simulink model "IEEE_BUS_68_Baseline"  (R2025a)
settings: Solver=ode23tb  StartTime=0.0  StopTime=150  FixedStep=Ts  MaxStep=0.0001  RelTol=1e-3
PreLoadFcn:
  | PSSMODEL=1;
  | LPSS=0;
  | WAPSS=0;
  | WAPSS2=0;
  | Ts=50e-5;
InitFcn:
  | PSSMODEL=1;
  | LPSS=0;
  | WAPSS=0;
  | WAPSS2=0;
  | Ts=50e-5;
  | 
  | % Required data to 68 Bus benchmark
  | % clear
  | % clc
  | % Definition for the columns
  | % system base =100 MVA
  | 
  | %% Line data Format (line)
  | % All values are given on the same system base MVA
  | % 1: From bus
  | % 2: To bus
  | % 3: Resistance (pu)
  | % 4: Reactance  (pu)
  | % 5: Charge     (pu)
  | % 6: Transformer Tap Amplitute
  | % 7: base MVA
  | % 8: Nomonal Voltage (KV)
  | 
  | %1   2    3        4       5       6        7      8
  | line=[...
  | 1	54	0	     0.0181	  0	      1.025     100    13.8
  | 2	58	0	     0.025	  0	      1.070     100    13.8
  | 3	62	0	     0.02	  0	      1.070     100    13.8
  | 4	19	0.0007	 0.0142	  0	      1.070     100    13.8
  | 5	20	0.0009	 0.018	  0	      1.009     100    13.8
  | 6	22	0	     0.0143	  0	      1.025     100    13.8
  | 7	23	0.0005	 0.0272	  0	      0         100    13.8
  | 8	25	0.0006	 0.0232	  0	      1.025     100    13.8
  | 9	29	0.0008	 0.0156   0	      1.025     100    13.8
  | 10	31	0	     0.026	  0	      1.04      100    13.8
  | 11	32	0	     0.013	  0	      1.04      100    13.8
  | 12	36	0	     0.0075	  0	      1.04      100    13.8
  | 13	17	0	     0.0033	  0	      1.04      100    13.8
  | 14	41	0	     0.0015	  0	      1         100    13.8
  | 15	42	0	     0.0015	  0	      1         100    13.8
  | 16	18	0	     0.003	  0	      1         100    13.8
  | 17	36	0.0005	 0.0045	  0.32	  0         100    138
  | 17	43	0.0005	 0.0276	  0	      0         100    138
  | 18	42	0.004	 0.06	  2.25    0         100    138
  | 18	49	0.0076	 0.1141	  1.16    0	        100    138
  | 18	50	0.0012	 0.0288	  2.06	  0         100    138
  | 20	19	0.0007	 0.0138	  0       1.06	    100    138
  | 19	68	0.0016	 0.0195	  0.304	  0         100    138
  | 21	22	0.0008	 0.014	  0.2565  0	        100    138
  | 21	68	0.0008	 0.0135	  0.2548  0	        100    138
  | 22	23	0.0006	 0.0096	  0.1846  0	        100    138
  | 23	24	0.0022	 0.035	  0.361	  0         100    138
  | 24	68	0.0003	 0.0059	  0.068	  0         100    138
  | 25	26	0.0032	 0.0323	  0.531	  0         100    138
  | 25	54	0.007	 0.0086	  0.146	  0         100    138
  | 26	27	0.0014	 0.0147	  0.2396  0	        100    138
  | 26	28	0.0043	 0.0474	  0.7802  0	        100    138
  | 26	29	0.0057	 0.0625	  1.029	  0         100    138
  | 27	37	0.0013	 0.0173	  0.3216  0	        100    138
  | 27	53	0.032	 0.32	  0.41	  0         100    138
  | ... (+206 lines)
undefined symbols (not defined in the file or in its folder): D1, Delta
libraries: spsRMSLib x73, spsThreePhaseVIMeasurementLib x69, spsLoadFlowBusLib x69, spsThreePhasePISectionLineLib x64, spsThreePhaseParallelRLCLoadLib x35, spsGenericPowerSystemStabilizerLib x32, spsThreePhaseSeriesRLCLoadLib x21, spsThreePhaseTransformerTwoWindingsLib x21, spsSynchronousMachinepuStandardLib x19, spsExcitationSystemLib x16, spsMultiBandPowerSystemStabilizerLib x16, spsSteamTurbineandGovernorLib x16
(part 6 of 7)

== system IEEE_BUS_68_Baseline/area-2/gen3/M3: Turbine & Regulators  ==
  note: M3
  m3 : Inport
  Pref3 : Inport  Port=2
  Vref3 : Inport  Port=3
  PSS3 : Inport  Port=4
  Bus Selector : BusSelector  OutputSignals="Mechanical.Rotor speed  wm  (pu),Mechanical.Rotor angle deviation  d_theta (rad),Mechanical.Electrical power  Pe (pu),Mechanical.Rotor speed deviation  dw (pu),Mechanical.Rotor mechanical angle  theta (deg),dq0 components.Stator voltage  vd (pu),dq0 components.Stator voltage  vq (pu),Output reactive power  Qeo (pu)"
  "Delta Pa PSS 3 " : spsGenericPowerSystemStabilizerLib/Generic Power System Stabilizer  Tsensor=15e-3  K=2.5*1.25  Twashout=1  Tleadlag1=[60e-3 1]  Tleadlag2=[0 0]  VSlimits=[-0.15 0.15]  Vinit=0  Plot_On=off  MagdB_On=on  FreqRange=logspace(-2,2,500)
      settings: LibrarySourceBlock=|
      | sps_lib/Electrical Machines/Synchronous Machine Control/Generic
      | Power System Stabilizer
  Delta w PSS (Kundur) 3 : spsGenericPowerSystemStabilizerLib/Generic Power System Stabilizer  Tsensor=15e-3  K=30  Twashout=10  Tleadlag1=[50e-3 20e-3]  Tleadlag2=[3 5.4]  VSlimits=[-0.15 0.15]  Vinit=0  Plot_On=off  MagdB_On=on  FreqRange=logspace(-2,2,500)
      settings: LibrarySourceBlock=|
      | sps_lib/Electrical Machines/Synchronous Machine Control/Generic
      | Power System Stabilizer
  EXCITATION3 : spsExcitationSystemLib/Excitation System  tr=AVR_Data(3,1)  reg=[ AVR_Data(3,2:3) ]  exc=[ 1, 0 ]  tgr=[ AVR_Data(3,4:5)]  damp=[ 0, 0 ]  sat=[ 0, 0 ]  lim="[ AVR_Data(3,7:8)  0 ]"  v0=[0.983 0.98901]
      settings: LibrarySourceBlock=sps_lib/Electrical Machines/Synchronous Machine Control/Excitation System
  MB-PSS3 : spsMultiBandPowerSystemStabilizerLib/Multi-Band Power System Stabilizer  OperationMode=Simplified settings  Kg=MB(1)  GL=[MB(2) MB(3)]  GI=[MB(4) MB(5)]  GH=[MB(6) MB(7)]  GLd=[66 66 9.4]  TcLF=[1.667 2 0 0 0 0 2 2.4 0 0 0 0 1 1]  GId=[66 66 47.6]  TcIF=[1 1 0.25 0.3 0 0 1 1 0.3 0.36 0 0 0 0]  GHd=[66 66 233]  TcHF="[0.01 0.012 0 0 0 0  0.012 0.0144 0 0 0 0 1 1]"  LIM=[.075 .15 .15 .15]  Plot_On=off  MagdB_On=off  FreqRange=logspace(-2,2,500)
      settings: LibrarySourceBlock=|
      | sps_lib/Electrical Machines/Synchronous Machine Control/Multi-Band
      | Power System Stabilizer
  Multiport Switch1 : MultiPortSwitch  Inputs=4  SaturateOnIntegerOverflow=off
  PSS model3 : Constant  Value=0
  PSS model4 : Constant
  Real-Imag to Complex1 : RealImagToComplex
  STG3 : spsSteamTurbineandGovernorLib/Steam Turbine and Governor  gentype=Tandem-compound (single mass)  reg1="[ 1  0.05    0 ]"  reg2="[ 0.001  0.15 ]"  reg3="[ -0.1  0.1  0  4.496 ]"  N=Ns  turb1="[ 0  10   3.3   0.5   ]"  turb2="[   0   0.36    0.36   0.28   ]"  HA="[ 0.046  1.430  1.465   0.192 ]"  KA="[ 90.44  53.88  64.59   62.94  ]"  DA="[ 0.0115  0.3575  0.3663   0.0137  ]"  ini1=0.325  ini2=[0.779316,-31.4247]
      settings: LibrarySourceBlock=|
      | sps_lib/Electrical Machines/Synchronous Machine Control/Steam Turbine
      | and Governor
  Sum2 : Sum  InputSameDT=on  SaturateOnIntegerOverflow=on  OutDataTypeStr=Inherit: Same as first input
  Sum3 : Sum  Inputs=-+  InputSameDT=on  SaturateOnIntegerOverflow=on  OutDataTypeStr=Inherit: Same as first input
  Terminator3 : Terminator
  Terminator4 : Terminator
  Terminator5 : Terminator
  wref3 : Constant
  Pm3 : Outport  InitialOutput=0
  Vf3 : Outport  Port=2  InitialOutput=0
  tag scope: EFD3=global, Pa3=global, Pe3=global, Q3=global, Vt3=global, d_theta3=global, pss3=global, theta3=global, w3=global
  wires:
  PSS3/1 -> Sum2/1
  Multiport Switch1/1 -> EXCITATION3/4, [pss3]
  PSS model3/1 -> Multiport Switch1/2
  MB-PSS3/1 -> Multiport Switch1/3
  Delta w PSS (Kundur) 3/1 -> Multiport Switch1/4
  "Delta Pa PSS 3 "/1 -> Multiport Switch1/5
  PSS model4/1 -> Sum2/2
  Sum2/1 -> Multiport Switch1/1
  Sum3/1 -> "Delta Pa PSS 3 "/1, [Pa3]  "Pm-Pe"
  Bus Selector/8 -> [Q3]  "<Output reactive power  Qeo (pu)>"
  Bus Selector/4 -> MB-PSS3/1, Delta w PSS (Kundur) 3/1  "<Rotor speed deviation  dw (pu)>"
  Bus Selector/3 -> [Pe3], Sum3/1  "<Electrical power  Pe (pu)>"
  Bus Selector/2 -> [d_theta3], STG3/4  "<Rotor angle deviation  d_theta (rad)>"
  Bus Selector/1 -> STG3/3, [w3]  "<Rotor speed  wm  (pu)>"
  STG3/1 -> Terminator5/1
  STG3/2 -> Terminator4/1
  STG3/4 -> Pm3/1, Sum3/2
  STG3/3 -> Terminator3/1
  Bus Selector/6 -> Real-Imag to Complex1/1, EXCITATION3/2  "<Stator voltage  vd (pu)>"
  Bus Selector/5 -> [theta3]  "<Rotor mechanical angle  theta (deg)>"
  Real-Imag to Complex1/1 -> [Vt3]
  EXCITATION3/1 -> [EFD3], Vf3/1
  Vref3/1 -> EXCITATION3/1
  m3/1 -> Bus Selector/1
  Pref3/1 -> STG3/2
  wref3/1 -> STG3/1
  Bus Selector/7 -> Real-Imag to Complex1/2, EXCITATION3/3  "<Stator voltage  vq (pu)>"

== system IEEE_BUS_68_Baseline/area-3/G1/M1: Turbine & Regulators  ==
  note: M1
  m1 : Inport
  Pref1 : Inport  Port=2
  Vref1 : Inport  Port=3
  PSS1 : Inport  Port=4
  Bus Selector : BusSelector  OutputSignals="Mechanical.Rotor speed  wm  (pu),Mechanical.Rotor angle deviation  d_theta (rad),Mechanical.Electrical power  Pe (pu),Mechanical.Rotor speed deviation  dw (pu),Mechanical.Rotor mechanical angle  theta (deg),dq0 components.Stator voltage  vd (pu),dq0 components.Stator voltage  vq (pu),Output reactive power  Qeo (pu)"
  "Delta Pa PSS 1 " : spsGenericPowerSystemStabilizerLib/Generic Power System Stabilizer  Tsensor=15e-3  K=2.5*1.25  Twashout=1  Tleadlag1=[60e-3 1]  Tleadlag2=[0 0]  VSlimits=[-0.15 0.15]  Vinit=0  Plot_On=off  MagdB_On=on  FreqRange=logspace(-2,2,500)
      settings: LibrarySourceBlock=|
      | sps_lib/Electrical Machines/Synchronous Machine Control/Generic
      | Power System Stabilizer
  Delta w PSS (Kundur) 1 : spsGenericPowerSystemStabilizerLib/Generic Power System Stabilizer  Tsensor=15e-3  K=30  Twashout=10  Tleadlag1=[50e-3 20e-3]  Tleadlag2=[3 5.4]  VSlimits=[-0.15 0.15]  Vinit=0  Plot_On=off  MagdB_On=on  FreqRange=logspace(-2,2,500)
      settings: LibrarySourceBlock=|
      | sps_lib/Electrical Machines/Synchronous Machine Control/Generic
      | Power System Stabilizer
  EXCITATION1 : spsExcitationSystemLib/Excitation System  tr=AVR_Data(1,1)  reg=[ AVR_Data(1,2:3) ]  exc=[ 1, 0 ]  tgr=[ AVR_Data(1,4:5)]  damp=[ 0, 0 ]  sat=[ 0, 0 ]  lim="[ AVR_Data(1,7:8)  0 ]"  v0=[1.045 1.06]
      settings: LibrarySourceBlock=sps_lib/Electrical Machines/Synchronous Machine Control/Excitation System
  MB-PSS1 : spsMultiBandPowerSystemStabilizerLib/Multi-Band Power System Stabilizer  OperationMode=Simplified settings  Kg=MB(1)  GL=[MB(2) MB(3)]  GI=[MB(4) MB(5)]  GH=[MB(6) MB(7)]  GLd=[66 66 9.4]  TcLF=[1.667 2 0 0 0 0 2 2.4 0 0 0 0 1 1]  GId=[66 66 47.6]  TcIF=[1 1 0.25 0.3 0 0 1 1 0.3 0.36 0 0 0 0]  GHd=[66 66 233]  TcHF="[0.01 0.012 0 0 0 0  0.012 0.0144 0 0 0 0 1 1]"  LIM=[.075 .15 .15 .15]  Plot_On=off  MagdB_On=off  FreqRange=logspace(-2,2,500)
      settings: LibrarySourceBlock=|
      | sps_lib/Electrical Machines/Synchronous Machine Control/Multi-Band
      | Power System Stabilizer
  Multiport Switch1 : MultiPortSwitch  Inputs=4  SaturateOnIntegerOverflow=off
  PSS model3 : Constant  Value=0
  PSS model4 : Constant
  Real-Imag to Complex1 : RealImagToComplex
  STG1 : spsSteamTurbineandGovernorLib/Steam Turbine and Governor  gentype=Tandem-compound (single mass)  reg1="[ 1  0.05    0 ]"  reg2="[ 0.001  0.15 ]"  reg3="[ -0.1  0.1  0  4.496 ]"  N=Ns  turb1="[ 0  10   3.3   0.5   ]"  turb2="[   0   0.36    0.36   0.28   ]"  HA="[ 0.046  1.430  1.465   0.192 ]"  KA="[ 90.44  53.88  64.59   62.94  ]"  DA="[ 0.0115  0.3575  0.3663   0.0137  ]"  ini1=0.25  ini2=[0.779316,-31.4247]
      settings: LibrarySourceBlock=|
      | sps_lib/Electrical Machines/Synchronous Machine Control/Steam Turbine
      | and Governor
  Sum2 : Sum  InputSameDT=on  SaturateOnIntegerOverflow=on  OutDataTypeStr=Inherit: Same as first input
  Sum3 : Sum  Inputs=-+  InputSameDT=on  SaturateOnIntegerOverflow=on  OutDataTypeStr=Inherit: Same as first input
  Terminator3 : Terminator
  Terminator4 : Terminator
  Terminator5 : Terminator
  wref1 : Constant
  Pm1 : Outport  InitialOutput=0
  Vf1 : Outport  Port=2  InitialOutput=0
  tag scope: EFD1=global, Pa1=global, Pe1=global, Q1=global, Vt1=global, d_theta1=global, pss1=global, theta1=global, w1=global
  wires:
  PSS1/1 -> Sum2/1
  Multiport Switch1/1 -> EXCITATION1/4, [pss1]
  PSS model3/1 -> Multiport Switch1/2
  MB-PSS1/1 -> Multiport Switch1/3
  Delta w PSS (Kundur) 1/1 -> Multiport Switch1/4
  "Delta Pa PSS 1 "/1 -> Multiport Switch1/5
  PSS model4/1 -> Sum2/2
  Sum2/1 -> Multiport Switch1/1
  Sum3/1 -> "Delta Pa PSS 1 "/1, [Pa1]  "Pm-Pe"
  Bus Selector/8 -> [Q1]  "<Output reactive power  Qeo (pu)>"
  Bus Selector/4 -> MB-PSS1/1, Delta w PSS (Kundur) 1/1  "<Rotor speed deviation  dw (pu)>"
  Bus Selector/3 -> [Pe1], Sum3/1  "<Electrical power  Pe (pu)>"
  Bus Selector/2 -> [d_theta1], STG1/4  "<Rotor angle deviation  d_theta (rad)>"
  Bus Selector/1 -> STG1/3, [w1]  "<Rotor speed  wm  (pu)>"
  STG1/1 -> Terminator5/1
  STG1/2 -> Terminator4/1
  STG1/4 -> Pm1/1, Sum3/2
  STG1/3 -> Terminator3/1
  Bus Selector/6 -> Real-Imag to Complex1/1, EXCITATION1/2  "<Stator voltage  vd (pu)>"
  Bus Selector/5 -> [theta1]  "<Rotor mechanical angle  theta (deg)>"
  Real-Imag to Complex1/1 -> [Vt1]
  EXCITATION1/1 -> [EFD1], Vf1/1
  Vref1/1 -> EXCITATION1/1
  m1/1 -> Bus Selector/1
  Pref1/1 -> STG1/2
  wref1/1 -> STG1/1
  Bus Selector/7 -> Real-Imag to Complex1/2, EXCITATION1/3  "<Stator voltage  vq (pu)>"

== system IEEE_BUS_68_Baseline/area-3/G8/M8: Turbine & Regulators  ==
  note: M8
  m8 : Inport
  Pref8 : Inport  Port=2
  Vref8 : Inport  Port=3
  PSS8 : Inport  Port=4
  Bus Selector : BusSelector  OutputSignals="Mechanical.Rotor speed  wm  (pu),Mechanical.Rotor angle deviation  d_theta (rad),Mechanical.Electrical power  Pe (pu),Mechanical.Rotor speed deviation  dw (pu),Mechanical.Rotor mechanical angle  theta (deg),dq0 components.Stator voltage  vd (pu),dq0 components.Stator voltage  vq (pu),Output reactive power  Qeo (pu)"
  "Delta Pa PSS 8 " : spsGenericPowerSystemStabilizerLib/Generic Power System Stabilizer  Tsensor=15e-3  K=2.5*1.25  Twashout=1  Tleadlag1=[60e-3 1]  Tleadlag2=[0 0]  VSlimits=[-0.15 0.15]  Vinit=0  Plot_On=off  MagdB_On=on  FreqRange=logspace(-2,2,500)
      settings: LibrarySourceBlock=|
      | sps_lib/Electrical Machines/Synchronous Machine Control/Generic
      | Power System Stabilizer
  Delta w PSS (Kundur) 8 : spsGenericPowerSystemStabilizerLib/Generic Power System Stabilizer  Tsensor=15e-3  K=30  Twashout=10  Tleadlag1=[50e-3 20e-3]  Tleadlag2=[3 5.4]  VSlimits=[-0.15 0.15]  Vinit=0  Plot_On=off  MagdB_On=on  FreqRange=logspace(-2,2,500)
      settings: LibrarySourceBlock=|
      | sps_lib/Electrical Machines/Synchronous Machine Control/Generic
      | Power System Stabilizer
  EXCITATION8 : spsExcitationSystemLib/Excitation System  tr=AVR_Data(8,1)  reg=[ AVR_Data(8,2:3) ]  exc=[ 1, 0 ]  tgr=[ AVR_Data(8,4:5)]  damp=[ 0, 0 ]  sat=[ 0, 0 ]  lim="[ AVR_Data(8,7:8)  0 ]"  v0=[1.03 1.0424]
      settings: LibrarySourceBlock=sps_lib/Electrical Machines/Synchronous Machine Control/Excitation System
  MB-PSS8 : spsMultiBandPowerSystemStabilizerLib/Multi-Band Power System Stabilizer  OperationMode=Simplified settings  Kg=MB(1)  GL=[MB(2) MB(3)]  GI=[MB(4) MB(5)]  GH=[MB(6) MB(7)]  GLd=[66 66 9.4]  TcLF=[1.667 2 0 0 0 0 2 2.4 0 0 0 0 1 1]  GId=[66 66 47.6]  TcIF=[1 1 0.25 0.3 0 0 1 1 0.3 0.36 0 0 0 0]  GHd=[66 66 233]  TcHF="[0.01 0.012 0 0 0 0  0.012 0.0144 0 0 0 0 1 1]"  LIM=[.075 .15 .15 .15]  Plot_On=off  MagdB_On=off  FreqRange=logspace(-2,2,500)
      settings: LibrarySourceBlock=|
      | sps_lib/Electrical Machines/Synchronous Machine Control/Multi-Band
      | Power System Stabilizer
  Multiport Switch1 : MultiPortSwitch  Inputs=4  SaturateOnIntegerOverflow=off
  PSS model3 : Constant  Value=0
  PSS model4 : Constant
  Real-Imag to Complex1 : RealImagToComplex
  STG8 : spsSteamTurbineandGovernorLib/Steam Turbine and Governor  gentype=Tandem-compound (single mass)  reg1="[ 1  0.05    0 ]"  reg2="[ 0.001  0.15 ]"  reg3="[ -0.1  0.1  0  4.496 ]"  N=Ns  turb1="[ 0  10   3.3   0.5   ]"  turb2="[   0   0.36    0.36   0.28   ]"  HA="[ 0.046  1.430  1.465   0.192 ]"  KA="[ 90.44  53.88  64.59   62.94  ]"  DA="[ 0.0115  0.3575  0.3663   0.0137  ]"  ini1=0.54  ini2=[0.779316,-31.4247]
      settings: LibrarySourceBlock=|
      | sps_lib/Electrical Machines/Synchronous Machine Control/Steam Turbine
      | and Governor
  Sum2 : Sum  InputSameDT=on  SaturateOnIntegerOverflow=on  OutDataTypeStr=Inherit: Same as first input
  Sum3 : Sum  Inputs=-+  InputSameDT=on  SaturateOnIntegerOverflow=on  OutDataTypeStr=Inherit: Same as first input
  Terminator3 : Terminator
  Terminator4 : Terminator
  Terminator5 : Terminator
  wref8 : Constant
  Pm8 : Outport  InitialOutput=0
  Vf8 : Outport  Port=2  InitialOutput=0
  tag scope: EFD8=global, Pa8=global, Pe8=global, Q8=global, Vt8=global, d_theta8=global, pss8=global, theta8=global, w8=global
  wires:
  Bus Selector/7 -> EXCITATION8/3, Real-Imag to Complex1/2  "<Stator voltage  vq (pu)>"
  wref8/1 -> STG8/1
  Pref8/1 -> STG8/2
  m8/1 -> Bus Selector/1
  Vref8/1 -> EXCITATION8/1
  EXCITATION8/1 -> Vf8/1, [EFD8]
  Real-Imag to Complex1/1 -> [Vt8]
  Bus Selector/5 -> [theta8]  "<Rotor mechanical angle  theta (deg)>"
  Bus Selector/6 -> EXCITATION8/2, Real-Imag to Complex1/1  "<Stator voltage  vd (pu)>"
  STG8/3 -> Terminator3/1
  STG8/4 -> Sum3/2, Pm8/1
  STG8/2 -> Terminator4/1
  STG8/1 -> Terminator5/1
  Bus Selector/1 -> [w8], STG8/3  "<Rotor speed  wm  (pu)>"
  Bus Selector/2 -> STG8/4, [d_theta8]  "<Rotor angle deviation  d_theta (rad)>"
  Bus Selector/3 -> Sum3/1, [Pe8]  "<Electrical power  Pe (pu)>"
  Bus Selector/4 -> Delta w PSS (Kundur) 8/1, MB-PSS8/1  "<Rotor speed deviation  dw (pu)>"
  Bus Selector/8 -> [Q8]  "<Output reactive power  Qeo (pu)>"
  Sum3/1 -> [Pa8], "Delta Pa PSS 8 "/1  "Pm-Pe"
  Sum2/1 -> Multiport Switch1/1
  PSS model4/1 -> Sum2/2
  "Delta Pa PSS 8 "/1 -> Multiport Switch1/5
  Delta w PSS (Kundur) 8/1 -> Multiport Switch1/4
  MB-PSS8/1 -> Multiport Switch1/3
  PSS model3/1 -> Multiport Switch1/2
  Multiport Switch1/1 -> [pss8], EXCITATION8/4
  PSS8/1 -> Sum2/1

== system IEEE_BUS_68_Baseline/area-3/G9/M9: Turbine & Regulators  ==
  note: M9
  m9 : Inport
  Pref9 : Inport  Port=2
  Vref9 : Inport  Port=3
  PSS9 : Inport  Port=4
  Bus Selector : BusSelector  OutputSignals="Mechanical.Rotor speed  wm  (pu),Mechanical.Rotor angle deviation  d_theta (rad),Mechanical.Electrical power  Pe (pu),Mechanical.Rotor speed deviation  dw (pu),Mechanical.Rotor mechanical angle  theta (deg),dq0 components.Stator voltage  vd (pu),dq0 components.Stator voltage  vq (pu),Output reactive power  Qeo (pu)"
  "Delta Pa PSS 9 " : spsGenericPowerSystemStabilizerLib/Generic Power System Stabilizer  Tsensor=15e-3  K=2.5*1.25  Twashout=1  Tleadlag1=[60e-3 1]  Tleadlag2=[0 0]  VSlimits=[-0.15 0.15]  Vinit=0  Plot_On=off  MagdB_On=on  FreqRange=logspace(-2,2,500)
      settings: LibrarySourceBlock=|
      | sps_lib/Electrical Machines/Synchronous Machine Control/Generic
      | Power System Stabilizer
  Delta w PSS (Kundur) 9 : spsGenericPowerSystemStabilizerLib/Generic Power System Stabilizer  Tsensor=15e-3  K=30  Twashout=10  Tleadlag1=[50e-3 20e-3]  Tleadlag2=[3 5.4]  VSlimits=[-0.15 0.15]  Vinit=0  Plot_On=off  MagdB_On=on  FreqRange=logspace(-2,2,500)
      settings: LibrarySourceBlock=|
      | sps_lib/Electrical Machines/Synchronous Machine Control/Generic
      | Power System Stabilizer
  EXCITATION9 : spsExcitationSystemLib/Excitation System  tr=AVR_Data(9,1)  reg=[ AVR_Data(9,2:3) ]  exc=[ 1, 0 ]  tgr=[ AVR_Data(9,4:5)]  damp=[ 0, 0 ]  sat=[ 0, 0 ]  lim="[ AVR_Data(9,7:8)  0 ]"  v0=[1.025 1.0447]
      settings: LibrarySourceBlock=sps_lib/Electrical Machines/Synchronous Machine Control/Excitation System
  MB-PSS9 : spsMultiBandPowerSystemStabilizerLib/Multi-Band Power System Stabilizer  OperationMode=Simplified settings  Kg=MB(1)  GL=[MB(2) MB(3)]  GI=[MB(4) MB(5)]  GH=[MB(6) MB(7)]  GLd=[66 66 9.4]  TcLF=[1.667 2 0 0 0 0 2 2.4 0 0 0 0 1 1]  GId=[66 66 47.6]  TcIF=[1 1 0.25 0.3 0 0 1 1 0.3 0.36 0 0 0 0]  GHd=[66 66 233]  TcHF="[0.01 0.012 0 0 0 0  0.012 0.0144 0 0 0 0 1 1]"  LIM=[.075 .15 .15 .15]  Plot_On=off  MagdB_On=off  FreqRange=logspace(-2,2,500)
      settings: LibrarySourceBlock=|
      | sps_lib/Electrical Machines/Synchronous Machine Control/Multi-Band
      | Power System Stabilizer
  Multiport Switch1 : MultiPortSwitch  Inputs=4  SaturateOnIntegerOverflow=off
  PSS model3 : Constant  Value=0
  PSS model4 : Constant
  Real-Imag to Complex1 : RealImagToComplex
  STG9 : spsSteamTurbineandGovernorLib/Steam Turbine and Governor  gentype=Tandem-compound (single mass)  reg1="[ 1  0.05    0 ]"  reg2="[ 0.001  0.15 ]"  reg3="[ -0.1  0.1  0  4.496 ]"  N=Ns  turb1="[ 0  10   3.3   0.5   ]"  turb2="[   0   0.36    0.36   0.28   ]"  HA="[ 0.046  1.430  1.465   0.192 ]"  KA="[ 90.44  53.88  64.59   62.94  ]"  DA="[ 0.0115  0.3575  0.3663   0.0137  ]"  ini1=0.8  ini2=[0.779316,-31.4247]
      settings: LibrarySourceBlock=|
      | sps_lib/Electrical Machines/Synchronous Machine Control/Steam Turbine
      | and Governor
  Sum2 : Sum  InputSameDT=on  SaturateOnIntegerOverflow=on  OutDataTypeStr=Inherit: Same as first input
  Sum3 : Sum  Inputs=-+  InputSameDT=on  SaturateOnIntegerOverflow=on  OutDataTypeStr=Inherit: Same as first input
  Terminator3 : Terminator
  Terminator4 : Terminator
  Terminator5 : Terminator
  wref9 : Constant
  Pm9 : Outport  InitialOutput=0
  Vf9 : Outport  Port=2  InitialOutput=0
  tag scope: EFD9=global, Pa9=global, Pe9=global, Q9=global, Vt9=global, d_theta9=global, pss9=global, theta9=global, w9=global
  wires:
  PSS9/1 -> Sum2/1
  Multiport Switch1/1 -> EXCITATION9/4, [pss9]
  PSS model3/1 -> Multiport Switch1/2
  MB-PSS9/1 -> Multiport Switch1/3
  Delta w PSS (Kundur) 9/1 -> Multiport Switch1/4
  "Delta Pa PSS 9 "/1 -> Multiport Switch1/5
  PSS model4/1 -> Sum2/2
  Sum2/1 -> Multiport Switch1/1
  Sum3/1 -> "Delta Pa PSS 9 "/1, [Pa9]  "Pm-Pe"
  Bus Selector/8 -> [Q9]  "<Output reactive power  Qeo (pu)>"
  Bus Selector/4 -> MB-PSS9/1, Delta w PSS (Kundur) 9/1  "<Rotor speed deviation  dw (pu)>"
  Bus Selector/3 -> [Pe9], Sum3/1  "<Electrical power  Pe (pu)>"
  Bus Selector/2 -> [d_theta9], STG9/4  "<Rotor angle deviation  d_theta (rad)>"
  Bus Selector/1 -> STG9/3, [w9]  "<Rotor speed  wm  (pu)>"
  STG9/1 -> Terminator5/1
  STG9/2 -> Terminator4/1
  STG9/4 -> Pm9/1, Sum3/2
  STG9/3 -> Terminator3/1
  Bus Selector/6 -> Real-Imag to Complex1/1, EXCITATION9/2  "<Stator voltage  vd (pu)>"
  Bus Selector/5 -> [theta9]  "<Rotor mechanical angle  theta (deg)>"
  Real-Imag to Complex1/1 -> [Vt9]
  EXCITATION9/1 -> [EFD9], Vf9/1
  Vref9/1 -> EXCITATION9/1
  m9/1 -> Bus Selector/1
  Pref9/1 -> STG9/2
  wref9/1 -> STG9/1
  Bus Selector/7 -> Real-Imag to Complex1/2, EXCITATION9/3  "<Stator voltage  vq (pu)>"

== system IEEE_BUS_68_Baseline/area-4/G10/M10: Turbine & Regulators  ==
  note: M10
  m10 : Inport
  Pref10 : Inport  Port=2
  Vref10 : Inport  Port=3
  PSS10 : Inport  Port=4
  Bus Selector : BusSelector  OutputSignals="Mechanical.Rotor speed  wm  (pu),Mechanical.Rotor angle deviation  d_theta (rad),Mechanical.Electrical power  Pe (pu),Mechanical.Rotor speed deviation  dw (pu),Mechanical.Rotor mechanical angle  theta (deg),dq0 components.Stator voltage  vd (pu),dq0 components.Stator voltage  vq (pu),Output reactive power  Qeo (pu)"
  "Delta Pa PSS 10 " : spsGenericPowerSystemStabilizerLib/Generic Power System Stabilizer  Tsensor=15e-3  K=2.5*1.25  Twashout=1  Tleadlag1=[60e-3 1]  Tleadlag2=[0 0]  VSlimits=[-0.15 0.15]  Vinit=0  Plot_On=off  MagdB_On=on  FreqRange=logspace(-2,2,500)
      settings: LibrarySourceBlock=|
      | sps_lib/Electrical Machines/Synchronous Machine Control/Generic
      | Power System Stabilizer
  Delta w PSS (Kundur) 10 : spsGenericPowerSystemStabilizerLib/Generic Power System Stabilizer  Tsensor=15e-3  K=30  Twashout=10  Tleadlag1=[50e-3 20e-3]  Tleadlag2=[3 5.4]  VSlimits=[-0.15 0.15]  Vinit=0  Plot_On=off  MagdB_On=on  FreqRange=logspace(-2,2,500)
      settings: LibrarySourceBlock=|
      | sps_lib/Electrical Machines/Synchronous Machine Control/Generic
      | Power System Stabilizer
  EXCITATION10 : spsExcitationSystemLib/Excitation System  tr=AVR_Data(7,1)  reg=[ AVR_Data(7,2:3) ]  exc=[ 1, 0 ]  tgr=[ AVR_Data(7,4:5)]  damp=[ 0, 0 ]  sat=[ 0, 0 ]  lim="[ AVR_Data(7,7:8)  0 ]"  v0=[1.01 1.0155]
      settings: LibrarySourceBlock=sps_lib/Electrical Machines/Synchronous Machine Control/Excitation System
  MB-PSS10 : spsMultiBandPowerSystemStabilizerLib/Multi-Band Power System Stabilizer  OperationMode=Simplified settings  Kg=MB(1)  GL=[MB(2) MB(3)]  GI=[MB(4) MB(5)]  GH=[MB(6) MB(7)]  GLd=[66 66 9.4]  TcLF=[1.667 2 0 0 0 0 2 2.4 0 0 0 0 1 1]  GId=[66 66 47.6]  TcIF=[1 1 0.25 0.3 0 0 1 1 0.3 0.36 0 0 0 0]  GHd=[66 66 233]  TcHF="[0.01 0.012 0 0 0 0  0.012 0.0144 0 0 0 0 1 1]"  LIM=[.075 .15 .15 .15]  Plot_On=off  MagdB_On=off  FreqRange=logspace(-2,2,500)
      settings: LibrarySourceBlock=|
      | sps_lib/Electrical Machines/Synchronous Machine Control/Multi-Band
      | Power System Stabilizer
  Multiport Switch1 : MultiPortSwitch  Inputs=4  SaturateOnIntegerOverflow=off
  PSS model3 : Constant  Value=0
  PSS model4 : Constant
  Real-Imag to Complex1 : RealImagToComplex
  STG10 : spsSteamTurbineandGovernorLib/Steam Turbine and Governor  gentype=Tandem-compound (single mass)  reg1="[ 1  0.05    0 ]"  reg2="[ 0.001  0.15 ]"  reg3="[ -0.1  0.1  0  4.496 ]"  N=Ns  turb1="[ 0  10   3.3   0.5   ]"  turb2="[   0   0.36    0.36   0.28   ]"  HA="[ 0.046  1.430  1.465   0.192 ]"  KA="[ 90.44  53.88  64.59   62.94  ]"  DA="[ 0.0115  0.3575  0.3663   0.0137  ]"  ini1=0.5  ini2=[0.779316,-31.4247]
      settings: LibrarySourceBlock=|
      | sps_lib/Electrical Machines/Synchronous Machine Control/Steam Turbine
      | and Governor
  Sum2 : Sum  InputSameDT=on  SaturateOnIntegerOverflow=on  OutDataTypeStr=Inherit: Same as first input
  Sum3 : Sum  Inputs=-+  InputSameDT=on  SaturateOnIntegerOverflow=on  OutDataTypeStr=Inherit: Same as first input
  Terminator3 : Terminator
  Terminator4 : Terminator
  Terminator5 : Terminator
  wref10 : Constant
  Pm10 : Outport  InitialOutput=0
  Vf10 : Outport  Port=2  InitialOutput=0
  tag scope: EFD10=global, Pa10=global, Pe10=global, Q10=global, Vt10=global, d_theta10=global, pss10=global, theta10=global, w10=global
  wires:
  PSS10/1 -> Sum2/1
  Multiport Switch1/1 -> EXCITATION10/4, [pss10]
  PSS model3/1 -> Multiport Switch1/2
  MB-PSS10/1 -> Multiport Switch1/3
  Delta w PSS (Kundur) 10/1 -> Multiport Switch1/4
  "Delta Pa PSS 10 "/1 -> Multiport Switch1/5
  PSS model4/1 -> Sum2/2
  Sum2/1 -> Multiport Switch1/1
  Sum3/1 -> "Delta Pa PSS 10 "/1, [Pa10]  "Pm-Pe"
  Bus Selector/8 -> [Q10]  "<Output reactive power  Qeo (pu)>"
  Bus Selector/4 -> MB-PSS10/1, Delta w PSS (Kundur) 10/1  "<Rotor speed deviation  dw (pu)>"
  Bus Selector/3 -> [Pe10], Sum3/1  "<Electrical power  Pe (pu)>"
  Bus Selector/2 -> [d_theta10], STG10/4  "<Rotor angle deviation  d_theta (rad)>"
  Bus Selector/1 -> STG10/3, [w10]  "<Rotor speed  wm  (pu)>"
  STG10/1 -> Terminator5/1
  STG10/2 -> Terminator4/1
  STG10/4 -> Pm10/1, Sum3/2
  STG10/3 -> Terminator3/1
  Bus Selector/6 -> Real-Imag to Complex1/1, EXCITATION10/2  "<Stator voltage  vd (pu)>"
  Bus Selector/5 -> [theta10]  "<Rotor mechanical angle  theta (deg)>"
  Real-Imag to Complex1/1 -> [Vt10]
  EXCITATION10/1 -> [EFD10], Vf10/1
  Vref10/1 -> EXCITATION10/1
  m10/1 -> Bus Selector/1
  Pref10/1 -> STG10/2
  wref10/1 -> STG10/1
  Bus Selector/7 -> Real-Imag to Complex1/2, EXCITATION10/3  "<Stator voltage  vq (pu)>"

== system IEEE_BUS_68_Baseline/area-4/G11/M11: Turbine & Regulators  ==
  note: M11
  m11 : Inport
  Pref11 : Inport  Port=2
  Vref11 : Inport  Port=3
  PSS11 : Inport  Port=4
  Bus Selector : BusSelector  OutputSignals="Mechanical.Rotor speed  wm  (pu),Mechanical.Rotor angle deviation  d_theta (rad),Mechanical.Electrical power  Pe (pu),Mechanical.Rotor speed deviation  dw (pu),Mechanical.Rotor mechanical angle  theta (deg),dq0 components.Stator voltage  vd (pu),dq0 components.Stator voltage  vq (pu),Output reactive power  Qeo (pu)"
  "Delta Pa PSS 11 " : spsGenericPowerSystemStabilizerLib/Generic Power System Stabilizer  Tsensor=15e-3  K=2.5*1.25  Twashout=1  Tleadlag1=[60e-3 1]  Tleadlag2=[0 0]  VSlimits=[-0.15 0.15]  Vinit=0  Plot_On=off  MagdB_On=on  FreqRange=logspace(-2,2,500)
      settings: LibrarySourceBlock=|
      | sps_lib/Electrical Machines/Synchronous Machine Control/Generic
      | Power System Stabilizer
  Delta w PSS (Kundur) 11 : spsGenericPowerSystemStabilizerLib/Generic Power System Stabilizer  Tsensor=15e-3  K=30  Twashout=10  Tleadlag1=[50e-3 20e-3]  Tleadlag2=[3 5.4]  VSlimits=[-0.15 0.15]  Vinit=0  Plot_On=off  MagdB_On=on  FreqRange=logspace(-2,2,500)
      settings: LibrarySourceBlock=|
      | sps_lib/Electrical Machines/Synchronous Machine Control/Generic
      | Power System Stabilizer
  EXCITATION11 : spsExcitationSystemLib/Excitation System  tr=AVR_Data(11,1)  reg=[ AVR_Data(11,2:3) ]  exc=[ 1, 0 ]  tgr=[ AVR_Data(11,4:5)]  damp=[ 0, 0 ]  sat=[ 0, 0 ]  lim="[ AVR_Data(11,7:8)  0 ]"  v0=[1 1.0051]
      settings: LibrarySourceBlock=sps_lib/Electrical Machines/Synchronous Machine Control/Excitation System
  MB-PSS11 : spsMultiBandPowerSystemStabilizerLib/Multi-Band Power System Stabilizer  OperationMode=Simplified settings  Kg=MB(1)  GL=[MB(2) MB(3)]  GI=[MB(4) MB(5)]  GH=[MB(6) MB(7)]  GLd=[66 66 9.4]  TcLF=[1.667 2 0 0 0 0 2 2.4 0 0 0 0 1 1]  GId=[66 66 47.6]  TcIF=[1 1 0.25 0.3 0 0 1 1 0.3 0.36 0 0 0 0]  GHd=[66 66 233]  TcHF="[0.01 0.012 0 0 0 0  0.012 0.0144 0 0 0 0 1 1]"  LIM=[.075 .15 .15 .15]  Plot_On=off  MagdB_On=off  FreqRange=logspace(-2,2,500)
      settings: LibrarySourceBlock=|
      | sps_lib/Electrical Machines/Synchronous Machine Control/Multi-Band
      | Power System Stabilizer
  Multiport Switch1 : MultiPortSwitch  Inputs=4  SaturateOnIntegerOverflow=off
  PSS model3 : Constant  Value=0
  PSS model4 : Constant
  Real-Imag to Complex1 : RealImagToComplex
  STG11 : spsSteamTurbineandGovernorLib/Steam Turbine and Governor  gentype=Tandem-compound (single mass)  reg1="[ 1  0.05    0 ]"  reg2="[ 0.001  0.15 ]"  reg3="[ -0.1  0.1  0  4.496 ]"  N=Ns  turb1="[ 0  10   3.3   0.5   ]"  turb2="[   0   0.36    0.36   0.28   ]"  HA="[ 0.046  1.430  1.465   0.192 ]"  KA="[ 90.44  53.88  64.59   62.94  ]"  DA="[ 0.0115  0.3575  0.3663   0.0137  ]"  ini1=0.5  ini2=[0.779316,-31.4247]
      settings: LibrarySourceBlock=|
      | sps_lib/Electrical Machines/Synchronous Machine Control/Steam Turbine
      | and Governor
  Sum2 : Sum  InputSameDT=on  SaturateOnIntegerOverflow=on  OutDataTypeStr=Inherit: Same as first input
  Sum3 : Sum  Inputs=-+  InputSameDT=on  SaturateOnIntegerOverflow=on  OutDataTypeStr=Inherit: Same as first input
  Terminator3 : Terminator
  Terminator4 : Terminator
  Terminator5 : Terminator
  wref11 : Constant
  Pm11 : Outport  InitialOutput=0
  Vf11 : Outport  Port=2  InitialOutput=0
  tag scope: EFD11=global, Pa11=global, Pe11=global, Q11=global, Vt11=global, d_theta11=global, pss11=global, theta11=global, w11=global
  wires:
  Bus Selector/7 -> EXCITATION11/3, Real-Imag to Complex1/2  "<Stator voltage  vq (pu)>"
  wref11/1 -> STG11/1
  Pref11/1 -> STG11/2
  m11/1 -> Bus Selector/1
  Vref11/1 -> EXCITATION11/1
  EXCITATION11/1 -> Vf11/1, [EFD11]
  Real-Imag to Complex1/1 -> [Vt11]
  Bus Selector/5 -> [theta11]  "<Rotor mechanical angle  theta (deg)>"
  Bus Selector/6 -> EXCITATION11/2, Real-Imag to Complex1/1  "<Stator voltage  vd (pu)>"
  STG11/3 -> Terminator3/1
  STG11/4 -> Sum3/2, Pm11/1
  STG11/2 -> Terminator4/1
  STG11/1 -> Terminator5/1
  Bus Selector/1 -> [w11], STG11/3  "<Rotor speed  wm  (pu)>"
  Bus Selector/2 -> STG11/4, [d_theta11]  "<Rotor angle deviation  d_theta (rad)>"
  Bus Selector/3 -> Sum3/1, [Pe11]  "<Electrical power  Pe (pu)>"
  Bus Selector/4 -> Delta w PSS (Kundur) 11/1, MB-PSS11/1  "<Rotor speed deviation  dw (pu)>"
  Bus Selector/8 -> [Q11]  "<Output reactive power  Qeo (pu)>"
  Sum3/1 -> [Pa11], "Delta Pa PSS 11 "/1  "Pm-Pe"
  Sum2/1 -> Multiport Switch1/1
  PSS model4/1 -> Sum2/2
  "Delta Pa PSS 11 "/1 -> Multiport Switch1/5
  Delta w PSS (Kundur) 11/1 -> Multiport Switch1/4
  MB-PSS11/1 -> Multiport Switch1/3
  PSS model3/1 -> Multiport Switch1/2
  Multiport Switch1/1 -> [pss11], EXCITATION11/4
  PSS11/1 -> Sum2/1

== system IEEE_BUS_68_Baseline/area-4/G12/M12: Turbine & Regulators  ==
  note: M12
  m12 : Inport
  Pref12 : Inport  Port=2
  Vref12 : Inport  Port=3
  PSS12 : Inport  Port=4
  Bus Selector : BusSelector  OutputSignals="Mechanical.Rotor speed  wm  (pu),Mechanical.Rotor angle deviation  d_theta (rad),Mechanical.Electrical power  Pe (pu),Mechanical.Rotor speed deviation  dw (pu),Mechanical.Rotor mechanical angle  theta (deg),dq0 components.Stator voltage  vd (pu),dq0 components.Stator voltage  vq (pu),Output reactive power  Qeo (pu)"
  "Delta Pa PSS 12 " : spsGenericPowerSystemStabilizerLib/Generic Power System Stabilizer  Tsensor=15e-3  K=2.5*1.25  Twashout=1  Tleadlag1=[60e-3 1]  Tleadlag2=[0 0]  VSlimits=[-0.15 0.15]  Vinit=0  Plot_On=off  MagdB_On=on  FreqRange=logspace(-2,2,500)
      settings: LibrarySourceBlock=|
      | sps_lib/Electrical Machines/Synchronous Machine Control/Generic
      | Power System Stabilizer
  Delta w PSS (Kundur) 12 : spsGenericPowerSystemStabilizerLib/Generic Power System Stabilizer  Tsensor=15e-3  K=30  Twashout=10  Tleadlag1=[50e-3 20e-3]  Tleadlag2=[3 5.4]  VSlimits=[-0.15 0.15]  Vinit=0  Plot_On=off  MagdB_On=on  FreqRange=logspace(-2,2,500)
      settings: LibrarySourceBlock=|
      | sps_lib/Electrical Machines/Synchronous Machine Control/Generic
      | Power System Stabilizer
  EXCITATION12 : spsExcitationSystemLib/Excitation System  tr=AVR_Data(13,1)  reg=[ AVR_Data(13,2:3) ]  exc=[ 1, 0 ]  tgr=[ AVR_Data(13,4:5)]  damp=[ 0, 0 ]  sat=[ 0, 0 ]  lim="[ AVR_Data(13,7:8)  0 ]"  v0=[1.0156 1.0134]
      settings: LibrarySourceBlock=sps_lib/Electrical Machines/Synchronous Machine Control/Excitation System
  MB-PSS12 : spsMultiBandPowerSystemStabilizerLib/Multi-Band Power System Stabilizer  OperationMode=Simplified settings  Kg=MB(1)  GL=[MB(2) MB(3)]  GI=[MB(4) MB(5)]  GH=[MB(6) MB(7)]  GLd=[66 66 9.4]  TcLF=[1.667 2 0 0 0 0 2 2.4 0 0 0 0 1 1]  GId=[66 66 47.6]  TcIF=[1 1 0.25 0.3 0 0 1 1 0.3 0.36 0 0 0 0]  GHd=[66 66 233]  TcHF="[0.01 0.012 0 0 0 0  0.012 0.0144 0 0 0 0 1 1]"  LIM=[.075 .15 .15 .15]  Plot_On=off  MagdB_On=off  FreqRange=logspace(-2,2,500)
      settings: LibrarySourceBlock=|
      | sps_lib/Electrical Machines/Synchronous Machine Control/Multi-Band
      | Power System Stabilizer
  Multiport Switch1 : MultiPortSwitch  Inputs=4  SaturateOnIntegerOverflow=off
  PSS model3 : Constant  Value=0
  PSS model4 : Constant
  Real-Imag to Complex1 : RealImagToComplex
  STG12 : spsSteamTurbineandGovernorLib/Steam Turbine and Governor  gentype=Tandem-compound (single mass)  reg1="[ 1  0.05    0 ]"  reg2="[ 0.001  0.15 ]"  reg3="[ -0.1  0.1  0  4.496 ]"  N=Ns  turb1="[ 0  10   3.3   0.5   ]"  turb2="[   0   0.36    0.36   0.28   ]"  HA="[ 0.046  1.430  1.465   0.192 ]"  KA="[ 90.44  53.88  64.59   62.94  ]"  DA="[ 0.0115  0.3575  0.3663   0.0137  ]"  ini1=0.45  ini2=[0.779316,-31.4247]
      settings: LibrarySourceBlock=|
      | sps_lib/Electrical Machines/Synchronous Machine Control/Steam Turbine
      | and Governor
  Sum2 : Sum  InputSameDT=on  SaturateOnIntegerOverflow=on  OutDataTypeStr=Inherit: Same as first input
  Sum3 : Sum  Inputs=-+  InputSameDT=on  SaturateOnIntegerOverflow=on  OutDataTypeStr=Inherit: Same as first input
  Terminator3 : Terminator
  Terminator4 : Terminator
  Terminator5 : Terminator
  wref12 : Constant
  Pm12 : Outport  InitialOutput=0
  Vf12 : Outport  Port=2  InitialOutput=0
  tag scope: EFD12=global, Pa12=global, Pe12=global, Q12=global, Vt12=global, d_theta12=global, pss12=global, theta12=global, w12=global
  wires:
  PSS12/1 -> Sum2/1
  Multiport Switch1/1 -> EXCITATION12/4, [pss12]
  PSS model3/1 -> Multiport Switch1/2
  MB-PSS12/1 -> Multiport Switch1/3
  Delta w PSS (Kundur) 12/1 -> Multiport Switch1/4
  "Delta Pa PSS 12 "/1 -> Multiport Switch1/5
  PSS model4/1 -> Sum2/2
  Sum2/1 -> Multiport Switch1/1
  Sum3/1 -> "Delta Pa PSS 12 "/1, [Pa12]  "Pm-Pe"
  Bus Selector/8 -> [Q12]  "<Output reactive power  Qeo (pu)>"
  Bus Selector/4 -> MB-PSS12/1, Delta w PSS (Kundur) 12/1  "<Rotor speed deviation  dw (pu)>"
  Bus Selector/3 -> [Pe12], Sum3/1  "<Electrical power  Pe (pu)>"
  Bus Selector/2 -> [d_theta12], STG12/4  "<Rotor angle deviation  d_theta (rad)>"
  Bus Selector/1 -> STG12/3, [w12]  "<Rotor speed  wm  (pu)>"
  STG12/1 -> Terminator5/1
  STG12/2 -> Terminator4/1
  STG12/4 -> Pm12/1, Sum3/2
  STG12/3 -> Terminator3/1
  Bus Selector/6 -> Real-Imag to Complex1/1, EXCITATION12/2  "<Stator voltage  vd (pu)>"
  Bus Selector/5 -> [theta12]  "<Rotor mechanical angle  theta (deg)>"
  Real-Imag to Complex1/1 -> [Vt12]
  EXCITATION12/1 -> [EFD12], Vf12/1
  Vref12/1 -> EXCITATION12/1
  m12/1 -> Bus Selector/1
  Pref12/1 -> STG12/2
  wref12/1 -> STG12/1
  Bus Selector/7 -> Real-Imag to Complex1/2, EXCITATION12/3  "<Stator voltage  vq (pu)>"

== system IEEE_BUS_68_Baseline/area-4/G13/M11: Turbine & Regulators  ==
  note: M13
  m13 : Inport
  Pref13 : Inport  Port=2
  Vref13 : Inport  Port=3
  PSS13 : Inport  Port=4
  Bus Selector : BusSelector  OutputSignals="Mechanical.Rotor speed  wm  (pu),Mechanical.Rotor angle deviation  d_theta (rad),Mechanical.Electrical power  Pe (pu),Mechanical.Rotor speed deviation  dw (pu),Mechanical.Rotor mechanical angle  theta (deg),dq0 components.Stator voltage  vd (pu),dq0 components.Stator voltage  vq (pu),Output reactive power  Qeo (pu)"
  "Delta Pa PSS 13 " : spsGenericPowerSystemStabilizerLib/Generic Power System Stabilizer  Tsensor=15e-3  K=2.5*1.25  Twashout=1  Tleadlag1=[60e-3 1]  Tleadlag2=[0 0]  VSlimits=[-0.15 0.15]  Vinit=0  Plot_On=off  MagdB_On=on  FreqRange=logspace(-2,2,500)
      settings: LibrarySourceBlock=|
      | sps_lib/Electrical Machines/Synchronous Machine Control/Generic
      | Power System Stabilizer
  Delta w PSS (Kundur) 13 : spsGenericPowerSystemStabilizerLib/Generic Power System Stabilizer  Tsensor=15e-3  K=30  Twashout=10  Tleadlag1=[50e-3 20e-3]  Tleadlag2=[3 5.4]  VSlimits=[-0.15 0.15]  Vinit=0  Plot_On=off  MagdB_On=on  FreqRange=logspace(-2,2,500)
      settings: LibrarySourceBlock=|
      | sps_lib/Electrical Machines/Synchronous Machine Control/Generic
      | Power System Stabilizer
  EXCITATION13 : spsExcitationSystemLib/Excitation System  tr=AVR_Data(13,1)  reg=[ AVR_Data(13,2:3) ]  exc=[ 1, 0 ]  tgr=[ AVR_Data(13,4:5)]  damp=[ 0, 0 ]  sat=[ 0, 0 ]  lim="[ AVR_Data(13,7:8)  0 ]"  v0=[1.011 1.0159]
      settings: LibrarySourceBlock=sps_lib/Electrical Machines/Synchronous Machine Control/Excitation System
  MB-PSS13 : spsMultiBandPowerSystemStabilizerLib/Multi-Band Power System Stabilizer  OperationMode=Simplified settings  Kg=MB(1)  GL=[MB(2) MB(3)]  GI=[MB(4) MB(5)]  GH=[MB(6) MB(7)]  GLd=[66 66 9.4]  TcLF=[1.667 2 0 0 0 0 2 2.4 0 0 0 0 1 1]  GId=[66 66 47.6]  TcIF=[1 1 0.25 0.3 0 0 1 1 0.3 0.36 0 0 0 0]  GHd=[66 66 233]  TcHF="[0.01 0.012 0 0 0 0  0.012 0.0144 0 0 0 0 1 1]"  LIM=[.075 .15 .15 .15]  Plot_On=off  MagdB_On=off  FreqRange=logspace(-2,2,500)
      settings: LibrarySourceBlock=|
      | sps_lib/Electrical Machines/Synchronous Machine Control/Multi-Band
      | Power System Stabilizer
  Multiport Switch1 : MultiPortSwitch  Inputs=4  SaturateOnIntegerOverflow=off
  PSS model3 : Constant  Value=0
  PSS model4 : Constant
  Real-Imag to Complex1 : RealImagToComplex
  STG13 : spsSteamTurbineandGovernorLib/Steam Turbine and Governor  gentype=Tandem-compound (single mass)  reg1="[ 1  0.05    0 ]"  reg2="[ 0.001  0.15 ]"  reg3="[ -0.1  0.1  0  4.496 ]"  N=Ns  turb1="[ 0  10   3.3   0.5   ]"  turb2="[   0   0.36    0.36   0.28   ]"  HA="[ 0.046  1.430  1.465   0.192 ]"  KA="[ 90.44  53.88  64.59   62.94  ]"  DA="[ 0.0115  0.3575  0.3663   0.0137  ]"  ini1=0.5985  ini2=[0.779316,-31.4247]
      settings: LibrarySourceBlock=|
      | sps_lib/Electrical Machines/Synchronous Machine Control/Steam Turbine
      | and Governor
  Sum2 : Sum  InputSameDT=on  SaturateOnIntegerOverflow=on  OutDataTypeStr=Inherit: Same as first input
  Sum3 : Sum  Inputs=-+  InputSameDT=on  SaturateOnIntegerOverflow=on  OutDataTypeStr=Inherit: Same as first input
  Terminator3 : Terminator
  Terminator4 : Terminator
  Terminator5 : Terminator
  wref13 : Constant
  Pm13 : Outport  InitialOutput=0
  Vf13 : Outport  Port=2  InitialOutput=0
  tag scope: EFD13=global, Pa13=global, Pe13=global, Q13=global, Vt13=global, d_theta13=global, pss13=global, theta13=global, w13=global
  wires:
  Bus Selector/7 -> EXCITATION13/3, Real-Imag to Complex1/2  "<Stator voltage  vq (pu)>"
  wref13/1 -> STG13/1
  Pref13/1 -> STG13/2
  m13/1 -> Bus Selector/1
  Vref13/1 -> EXCITATION13/1
  EXCITATION13/1 -> Vf13/1, [EFD13]
  Real-Imag to Complex1/1 -> [Vt13]
  Bus Selector/5 -> [theta13]  "<Rotor mechanical angle  theta (deg)>"
  Bus Selector/6 -> EXCITATION13/2, Real-Imag to Complex1/1  "<Stator voltage  vd (pu)>"
  STG13/3 -> Terminator3/1
  STG13/4 -> Sum3/2, Pm13/1
  STG13/2 -> Terminator4/1
  STG13/1 -> Terminator5/1
  Bus Selector/1 -> [w13], STG13/3  "<Rotor speed  wm  (pu)>"
  Bus Selector/2 -> STG13/4, [d_theta13]  "<Rotor angle deviation  d_theta (rad)>"
  Bus Selector/3 -> Sum3/1, [Pe13]  "<Electrical power  Pe (pu)>"
  Bus Selector/4 -> Delta w PSS (Kundur) 13/1, MB-PSS13/1  "<Rotor speed deviation  dw (pu)>"
  Bus Selector/8 -> [Q13]  "<Output reactive power  Qeo (pu)>"
  Sum3/1 -> [Pa13], "Delta Pa PSS 13 "/1  "Pm-Pe"
  Sum2/1 -> Multiport Switch1/1
  PSS model4/1 -> Sum2/2
  "Delta Pa PSS 13 "/1 -> Multiport Switch1/5
  Delta w PSS (Kundur) 13/1 -> Multiport Switch1/4
  MB-PSS13/1 -> Multiport Switch1/3
  PSS model3/1 -> Multiport Switch1/2
  Multiport Switch1/1 -> [pss13], EXCITATION13/4
  PSS13/1 -> Sum2/1

== system IEEE_BUS_68_Baseline/area-5/G14/M14: Turbine & Regulators  ==
  note: M14
  m14 : Inport
  Pref14 : Inport  Port=2
  Vref14 : Inport  Port=3
  PSS14 : Inport  Port=4
  Bus Selector : BusSelector  OutputSignals="Mechanical.Rotor speed  wm  (pu),Mechanical.Rotor angle deviation  d_theta (rad),Mechanical.Electrical power  Pe (pu),Mechanical.Rotor speed deviation  dw (pu),Mechanical.Rotor mechanical angle  theta (deg),dq0 components.Stator voltage  vd (pu),dq0 components.Stator voltage  vq (pu),Output reactive power  Qeo (pu)"
  "Delta Pa PSS 14 " : spsGenericPowerSystemStabilizerLib/Generic Power System Stabilizer  Tsensor=15e-3  K=2.5*1.25  Twashout=1  Tleadlag1=[60e-3 1]  Tleadlag2=[0 0]  VSlimits=[-0.15 0.15]  Vinit=0  Plot_On=off  MagdB_On=on  FreqRange=logspace(-2,2,500)
      settings: LibrarySourceBlock=|
      | sps_lib/Electrical Machines/Synchronous Machine Control/Generic
      | Power System Stabilizer
  Delta w PSS (Kundur) 14 : spsGenericPowerSystemStabilizerLib/Generic Power System Stabilizer  Tsensor=15e-3  K=30  Twashout=10  Tleadlag1=[50e-3 20e-3]  Tleadlag2=[3 5.4]  VSlimits=[-0.15 0.15]  Vinit=0  Plot_On=off  MagdB_On=on  FreqRange=logspace(-2,2,500)
      settings: LibrarySourceBlock=|
      | sps_lib/Electrical Machines/Synchronous Machine Control/Generic
      | Power System Stabilizer
  EXCITATION14 : spsExcitationSystemLib/Excitation System  tr=AVR_Data(14,1)  reg=[ AVR_Data(14,2:3) ]  exc=[ 1, 0 ]  tgr=[ AVR_Data(14,4:5)]  damp=[ 0, 0 ]  sat=[ 0, 0 ]  lim="[ AVR_Data(14,7:8)  0 ]"  v0=[1 1.0005]
      settings: LibrarySourceBlock=sps_lib/Electrical Machines/Synchronous Machine Control/Excitation System
  MB-PSS14 : spsMultiBandPowerSystemStabilizerLib/Multi-Band Power System Stabilizer  OperationMode=Simplified settings  Kg=MB(1)  GL=[MB(2) MB(3)]  GI=[MB(4) MB(5)]  GH=[MB(6) MB(7)]  GLd=[66 66 9.4]  TcLF=[1.667 2 0 0 0 0 2 2.4 0 0 0 0 1 1]  GId=[66 66 47.6]  TcIF=[1 1 0.25 0.3 0 0 1 1 0.3 0.36 0 0 0 0]  GHd=[66 66 233]  TcHF="[0.01 0.012 0 0 0 0  0.012 0.0144 0 0 0 0 1 1]"  LIM=[.075 .15 .15 .15]  Plot_On=off  MagdB_On=off  FreqRange=logspace(-2,2,500)
      settings: LibrarySourceBlock=|
      | sps_lib/Electrical Machines/Synchronous Machine Control/Multi-Band
      | Power System Stabilizer
  Multiport Switch1 : MultiPortSwitch  Inputs=4  SaturateOnIntegerOverflow=off
  PSS model3 : Constant  Value=0
  PSS model4 : Constant
  Real-Imag to Complex1 : RealImagToComplex
  STG14 : spsSteamTurbineandGovernorLib/Steam Turbine and Governor  gentype=Tandem-compound (single mass)  reg1="[ 1  0.05    0 ]"  reg2="[ 0.001  0.15 ]"  reg3="[ -0.1  0.1  0  4.496 ]"  N=Ns  turb1="[ 0  10   3.3   0.5   ]"  turb2="[   0   0.36    0.36   0.28   ]"  HA="[ 0.046  1.430  1.465   0.192 ]"  KA="[ 90.44  53.88  64.59   62.94  ]"  DA="[ 0.0115  0.3575  0.3663   0.0137  ]"  ini1=0.595  ini2=[0.779316,-31.4247]
      settings: LibrarySourceBlock=|
      | sps_lib/Electrical Machines/Synchronous Machine Control/Steam Turbine
      | and Governor
  Sum2 : Sum  InputSameDT=on  SaturateOnIntegerOverflow=on  OutDataTypeStr=Inherit: Same as first input
  Sum3 : Sum  Inputs=-+  InputSameDT=on  SaturateOnIntegerOverflow=on  OutDataTypeStr=Inherit: Same as first input
  Terminator3 : Terminator
  Terminator4 : Terminator
  Terminator5 : Terminator
  wref14 : Constant
  Pm14 : Outport  InitialOutput=0
  Vf14 : Outport  Port=2  InitialOutput=0
  tag scope: EFD14=global, Pa14=global, Pe14=global, Q14=global, Vt14=global, d_theta14=global, pss14=global, theta14=global, w14=global
  wires:
  PSS14/1 -> Sum2/1
  Multiport Switch1/1 -> EXCITATION14/4, [pss14]
  PSS model3/1 -> Multiport Switch1/2
  MB-PSS14/1 -> Multiport Switch1/3
  Delta w PSS (Kundur) 14/1 -> Multiport Switch1/4
  "Delta Pa PSS 14 "/1 -> Multiport Switch1/5
  PSS model4/1 -> Sum2/2
  Sum2/1 -> Multiport Switch1/1
  Sum3/1 -> "Delta Pa PSS 14 "/1, [Pa14]  "Pm-Pe"
  Bus Selector/8 -> [Q14]  "<Output reactive power  Qeo (pu)>"
  Bus Selector/4 -> MB-PSS14/1, Delta w PSS (Kundur) 14/1  "<Rotor speed deviation  dw (pu)>"
  Bus Selector/3 -> [Pe14], Sum3/1  "<Electrical power  Pe (pu)>"
  Bus Selector/2 -> [d_theta14], STG14/4  "<Rotor angle deviation  d_theta (rad)>"
  Bus Selector/1 -> STG14/3, [w14]  "<Rotor speed  wm  (pu)>"
  STG14/1 -> Terminator5/1
  STG14/2 -> Terminator4/1
  STG14/4 -> Pm14/1, Sum3/2
  STG14/3 -> Terminator3/1
  Bus Selector/6 -> Real-Imag to Complex1/1, EXCITATION14/2  "<Stator voltage  vd (pu)>"
  Bus Selector/5 -> [theta14]  "<Rotor mechanical angle  theta (deg)>"
  Real-Imag to Complex1/1 -> [Vt14]
  EXCITATION14/1 -> [EFD14], Vf14/1
  Vref14/1 -> EXCITATION14/1
  m14/1 -> Bus Selector/1
  Pref14/1 -> STG14/2
  wref14/1 -> STG14/1
  Bus Selector/7 -> Real-Imag to Complex1/2, EXCITATION14/3  "<Stator voltage  vq (pu)>"
